simulink model "ASM_Traffic_new"  (R2024a)
settings: Solver=ode1  StartTime=SIM.tstart.v  StopTime=SIM.tend.v  FixedStep=SIM.StepSize.v  RelTol=1e-3
PostLoadFcn:
  | if any(exist('dsrtsu_mdlpostloadfcn', 'file') ~= 0), dsrtsu_mdlpostloadfcn('Execute', bdroot); end
  | try, asm_mdl_postloadfcn(bdroot, 'UpdateModel', 3600); catch, disp(lasterr); end,
InitFcn:
  | , if any(exist('rtifpga_mdlclblib', 'file') ~= 0), rtifpga_mdlclblib('Init', bdroot); end,
  | , if any(exist('dsmpb_private', 'file') ~= 0), dsmpb_private('dsmpb_mdlclblib', 'Init', bdroot); end,
undefined symbols (not defined in the file): _to_, a0b2, ASM_BrakeHydraulics_DemoSystems, ASM_VehicleDynamics_DemoSystems, b98103fe8ad365046cd0, BrakeCircuit, CPT, Crankshaft, DiscIntNeverNeededParam, dsmsi, FinalDriveAssembly, MDL, ModeSignals, Pos_BrakePedal_Maneuver, rad, RefSignals, s_to_rpm, SIM, SoftECU, Suspension, Tire, Transmission
libraries: ASM_Traffic_lib x135, simulink x100, ASM_Utils_lib x77, ASM_VehicleDynamics_lib x70, ASM_Environment_lib x22, dsmpblib x20, dsmsilib x15, MDLD_Utils_lib x10, ASM_BrakeHydraulics_lib x3
(part 37 of 63)

== system ASM_Traffic_new/Environment/GroundTruth/UserInterface/PAR_Plant/Fellow_Vehicles ==
  Interface_In : Inport
  Bus Creator3 : BusCreator  Inputs=10
  Bus Creator4 : BusCreator  Inputs=1
  Bus Selector : BusSelector  OutputSignals=UserSignals_Customized.Fellow1_TurnLights
  Bus Selector1 : BusSelector  OutputSignals=UserSignals_Customized.Fellow2_TurnLights
  Bus Selector10 : BusSelector  OutputSignals=UserSignals_Customized.Fellow11_TurnLights
  Bus Selector11 : BusSelector  OutputSignals=UserSignals_Customized.Fellow12_TurnLights
  Bus Selector12 : BusSelector  OutputSignals=UserSignals_Customized.Fellow13_TurnLights
  Bus Selector13 : BusSelector  OutputSignals=UserSignals_Customized.Fellow14_TurnLights
  Bus Selector14 : BusSelector  OutputSignals=UserSignals_Customized.Fellow15_TurnLights
  Bus Selector15 : BusSelector  OutputSignals=UserSignals_Customized.Fellow16_TurnLights
  Bus Selector16 : BusSelector  OutputSignals=UserSignals_Customized.Fellow17_TurnLights
  Bus Selector17 : BusSelector  OutputSignals=UserSignals_Customized.Fellow18_TurnLights
  Bus Selector18 : BusSelector  OutputSignals=UserSignals_Customized.Fellow19_TurnLights
  Bus Selector19 : BusSelector  OutputSignals=UserSignals_Customized.Fellow20_TurnLights
  Bus Selector2 : BusSelector  OutputSignals=UserSignals_Customized.Fellow3_TurnLights
  Bus Selector20 : BusSelector  OutputSignals=UserSignals_Customized.Fellow21_TurnLights
  Bus Selector21 : BusSelector  OutputSignals=UserSignals_Customized.Fellow22_TurnLights
  Bus Selector22 : BusSelector  OutputSignals=UserSignals_Customized.Fellow23_TurnLights
  Bus Selector23 : BusSelector  OutputSignals=UserSignals_Customized.Fellow24_TurnLights
  Bus Selector24 : BusSelector  OutputSignals=UserSignals_Customized.Fellow25_TurnLights
  Bus Selector25 : BusSelector  OutputSignals=UserSignals_Customized.Fellow26_TurnLights
  Bus Selector26 : BusSelector  OutputSignals=UserSignals_Customized.Fellow27_TurnLights
  Bus Selector27 : BusSelector  OutputSignals=UserSignals_Customized.Fellow28_TurnLights
  Bus Selector28 : BusSelector  OutputSignals=UserSignals_Customized.Fellow29_TurnLights
  Bus Selector29 : BusSelector  OutputSignals=UserSignals_Customized.Fellow30_TurnLights
  Bus Selector3 : BusSelector  OutputSignals=UserSignals_Customized.Fellow4_TurnLights
  Bus Selector3000 : BusSelector  OutputSignals=Traffic.Plant.Traffic_Signals_toEnvironment
  Bus Selector4 : BusSelector  OutputSignals=UserSignals_Customized.Fellow5_TurnLights
  Bus Selector5 : BusSelector  OutputSignals=UserSignals_Customized.Fellow6_TurnLights
  Bus Selector6 : BusSelector  OutputSignals=UserSignals_Customized.Fellow7_TurnLights
  Bus Selector7 : BusSelector  OutputSignals=UserSignals_Customized.Fellow8_TurnLights
  Bus Selector8 : BusSelector  OutputSignals=UserSignals_Customized.Fellow9_TurnLights
  Bus Selector9 : BusSelector  OutputSignals=UserSignals_Customized.Fellow10_TurnLights
  Demux_Fellow_Lightstates : Subsystem
  Lightstates_Fellow1 : Subsystem
  Lightstates_Fellow10 : Subsystem
  Lightstates_Fellow11 : Subsystem
  Lightstates_Fellow12 : Subsystem
  Lightstates_Fellow13 : Subsystem
  Lightstates_Fellow14 : Subsystem
  Lightstates_Fellow15 : Subsystem
  Lightstates_Fellow16 : Subsystem
  Lightstates_Fellow17 : Subsystem
  Lightstates_Fellow18 : Subsystem
  Lightstates_Fellow19 : Subsystem
  Lightstates_Fellow2 : Subsystem
  Lightstates_Fellow20 : Subsystem
  Lightstates_Fellow21 : Subsystem
  Lightstates_Fellow22 : Subsystem
  Lightstates_Fellow23 : Subsystem
  Lightstates_Fellow24 : Subsystem
  Lightstates_Fellow25 : Subsystem
  Lightstates_Fellow26 : Subsystem
  Lightstates_Fellow27 : Subsystem
  Lightstates_Fellow28 : Subsystem
  Lightstates_Fellow29 : Subsystem
  Lightstates_Fellow3 : Subsystem
  Lightstates_Fellow30 : Subsystem
  Lightstates_Fellow4 : Subsystem
  Lightstates_Fellow5 : Subsystem
  Lightstates_Fellow6 : Subsystem
  Lightstates_Fellow7 : Subsystem
  Lightstates_Fellow8 : Subsystem
  Lightstates_Fellow9 : Subsystem
  Mux : Mux  Inputs=MDL.Traffic.MaxNumFellows.v
  Fellow_Vehicles[] : Outport  VectorParamsAs1DForOutWhenUnconnected=off
  wires:
  Bus Selector29/1 -> Lightstates_Fellow30/1(Fellow_Indicator_State[])  "<Fellow30_TurnLights>"
  Bus Selector28/1 -> Lightstates_Fellow29/1(Fellow_Indicator_State[])  "<Fellow29_TurnLights>"
  Bus Selector27/1 -> Lightstates_Fellow28/1(Fellow_Indicator_State[])  "<Fellow28_TurnLights>"
  Bus Selector26/1 -> Lightstates_Fellow27/1(Fellow_Indicator_State[])  "<Fellow27_TurnLights>"
  Bus Selector25/1 -> Lightstates_Fellow26/1(Fellow_Indicator_State[])  "<Fellow26_TurnLights>"
  Bus Selector24/1 -> Lightstates_Fellow25/1(Fellow_Indicator_State[])  "<Fellow25_TurnLights>"
  Bus Selector23/1 -> Lightstates_Fellow24/1(Fellow_Indicator_State[])  "<Fellow24_TurnLights>"
  Bus Selector22/1 -> Lightstates_Fellow23/1(Fellow_Indicator_State[])  "<Fellow23_TurnLights>"
  Bus Selector21/1 -> Lightstates_Fellow22/1(Fellow_Indicator_State[])  "<Fellow22_TurnLights>"
  Bus Selector20/1 -> Lightstates_Fellow21/1(Fellow_Indicator_State[])  "<Fellow21_TurnLights>"
  Bus Selector19/1 -> Lightstates_Fellow20/1(Fellow_Indicator_State[])  "<Fellow20_TurnLights>"
  Bus Selector18/1 -> Lightstates_Fellow19/1(Fellow_Indicator_State[])  "<Fellow19_TurnLights>"
  Bus Selector17/1 -> Lightstates_Fellow18/1(Fellow_Indicator_State[])  "<Fellow18_TurnLights>"
  Bus Selector16/1 -> Lightstates_Fellow17/1(Fellow_Indicator_State[])  "<Fellow17_TurnLights>"
  Bus Selector15/1 -> Lightstates_Fellow16/1(Fellow_Indicator_State[])  "<Fellow16_TurnLights>"
  Bus Selector14/1 -> Lightstates_Fellow15/1(Fellow_Indicator_State[])  "<Fellow15_TurnLights>"
  Bus Selector13/1 -> Lightstates_Fellow14/1(Fellow_Indicator_State[])  "<Fellow14_TurnLights>"
  Bus Selector12/1 -> Lightstates_Fellow13/1(Fellow_Indicator_State[])  "<Fellow13_TurnLights>"
  Bus Selector11/1 -> Lightstates_Fellow12/1(Fellow_Indicator_State[])  "<Fellow12_TurnLights>"
  Bus Selector10/1 -> Lightstates_Fellow11/1(Fellow_Indicator_State[])  "<Fellow11_TurnLights>"
  Bus Selector9/1 -> Lightstates_Fellow10/1(Fellow_Indicator_State[])  "<Fellow10_TurnLights>"
  Bus Selector8/1 -> Lightstates_Fellow9/1(Fellow_Indicator_State[])  "<Fellow9_TurnLights>"
  Bus Selector7/1 -> Lightstates_Fellow8/1(Fellow_Indicator_State[])  "<Fellow8_TurnLights>"
  Bus Selector6/1 -> Lightstates_Fellow7/1(Fellow_Indicator_State[])  "<Fellow7_TurnLights>"
  Bus Selector5/1 -> Lightstates_Fellow6/1(Fellow_Indicator_State[])  "<Fellow6_TurnLights>"
  Bus Selector4/1 -> Lightstates_Fellow5/1(Fellow_Indicator_State[])  "<Fellow5_TurnLights>"
  Bus Selector3/1 -> Lightstates_Fellow4/1(Fellow_Indicator_State[])  "<Fellow4_TurnLights>"
  Bus Selector2/1 -> Lightstates_Fellow3/1(Fellow_Indicator_State[])  "<Fellow3_TurnLights>"
  Bus Selector1/1 -> Lightstates_Fellow2/1(Fellow_Indicator_State[])  "<Fellow2_TurnLights>"
  Bus Selector/1 -> Lightstates_Fellow1/1(Fellow_Indicator_State[])  "<Fellow1_TurnLights>"
  Bus Selector3000/1 -> Bus Selector1/1, Bus Selector2/1, Bus Selector3/1, Bus Selector4/1, Bus Selector5/1, Bus Selector6/1, Bus Selector7/1, Bus Selector8/1, Bus Selector9/1, Bus Selector10/1, Bus Selector11/1, Bus Selector12/1, Bus Selector13/1, Bus Selector14/1, Bus Selector15/1, Bus Selector16/1, Bus Selector17/1, Bus Selector18/1, Bus Selector19/1, Bus Selector20/1, Bus Selector21/1, Bus Selector22/1, Bus Selector23/1, Bus Selector24/1, Bus Selector25/1, Bus Selector26/1, Bus Selector27/1, Bus Selector28/1, Bus Selector29/1, Bus Selector/1  "<Traffic_Signals_toEnvironment>"
  Lightstates_Fellow30/1(Lightstates[]) -> Mux/30
  Lightstates_Fellow29/1(Lightstates[]) -> Mux/29
  Lightstates_Fellow28/1(Lightstates[]) -> Mux/28
  Lightstates_Fellow27/1(Lightstates[]) -> Mux/27
  Lightstates_Fellow26/1(Lightstates[]) -> Mux/26
  Lightstates_Fellow25/1(Lightstates[]) -> Mux/25
  Lightstates_Fellow24/1(Lightstates[]) -> Mux/24
  Lightstates_Fellow23/1(Lightstates[]) -> Mux/23
  Lightstates_Fellow22/1(Lightstates[]) -> Mux/22
  Lightstates_Fellow21/1(Lightstates[]) -> Mux/21
  Lightstates_Fellow20/1(Lightstates[]) -> Mux/20
  Lightstates_Fellow19/1(Lightstates[]) -> Mux/19
  Lightstates_Fellow18/1(Lightstates[]) -> Mux/18
  Lightstates_Fellow17/1(Lightstates[]) -> Mux/17
  Lightstates_Fellow16/1(Lightstates[]) -> Mux/16
  Lightstates_Fellow1/1(Lightstates[]) -> Mux/1
  Lightstates_Fellow2/1(Lightstates[]) -> Mux/2
  Lightstates_Fellow3/1(Lightstates[]) -> Mux/3
  Lightstates_Fellow4/1(Lightstates[]) -> Mux/4
  Lightstates_Fellow5/1(Lightstates[]) -> Mux/5
  Lightstates_Fellow6/1(Lightstates[]) -> Mux/6
  Lightstates_Fellow7/1(Lightstates[]) -> Mux/7
  Lightstates_Fellow8/1(Lightstates[]) -> Mux/8
  Lightstates_Fellow9/1(Lightstates[]) -> Mux/9
  Lightstates_Fellow10/1(Lightstates[]) -> Mux/10
  Lightstates_Fellow11/1(Lightstates[]) -> Mux/11
  Lightstates_Fellow12/1(Lightstates[]) -> Mux/12
  Lightstates_Fellow13/1(Lightstates[]) -> Mux/13
  Lightstates_Fellow14/1(Lightstates[]) -> Mux/14
  Lightstates_Fellow15/1(Lightstates[]) -> Mux/15
  Mux/1 -> Demux_Fellow_Lightstates/1(Fellow_Lightstates[])
  Bus Creator3/1 -> Bus Creator4/1  "Fellow_Vehicles_LightStates"
  Bus Creator4/1 -> Fellow_Vehicles[]/1  "Fellow_Vehicles[]"
  Demux_Fellow_Lightstates/10(Brake_Fellows[]) -> Bus Creator3/10  "Brake_Light[]"
  Demux_Fellow_Lightstates/9(Indicator_State_Fellows[]) -> Bus Creator3/9  "Indicator_State[]"
  Demux_Fellow_Lightstates/6(Rear_Fog_Light_Fellows[]) -> Bus Creator3/6  "Rear_Fog_Light[]"
  Demux_Fellow_Lightstates/5(License_Plate_Illumination_Fellows[]) -> Bus Creator3/5  "License_Plate_Illumination[]"
  Demux_Fellow_Lightstates/1(High_Beam_Fellows[]) -> Bus Creator3/1  "High_Beam[]"
  Demux_Fellow_Lightstates/2(Reversing_Light_Fellows[]) -> Bus Creator3/2  "Reversing_Light[]"
  Demux_Fellow_Lightstates/3(Front_Fog_Light_Fellows[]) -> Bus Creator3/3  "Front_Fog_Light[]"
  Demux_Fellow_Lightstates/4(Head_Light_Fellows[]) -> Bus Creator3/4  "Head_Light[]"
  Demux_Fellow_Lightstates/7(Emergency_Veh_Illu_Fellows[]) -> Bus Creator3/7  "Emergency_Veh_Illu_Fellows[]"
  Demux_Fellow_Lightstates/8(Service_Veh_Illu_Fellows[]) -> Bus Creator3/8  "Service_Veh_Illu_Fellows[]"
  Interface_In/1 -> Bus Selector3000/1

== system ASM_Traffic_new/Environment/GroundTruth/UserInterface/PAR_Plant/HostVehicle_Data_AutomatedDrivingFunction ==
  Interface_In : Inport
  AutomatedDrivingFunction_1 : Subsystem
  AutomatedDrivingFunction_2 : Subsystem
  AutomatedDrivingFunction_3 : Subsystem
  AutomatedDrivingFunction_4 : Subsystem
  Bus Creator : BusCreator  Inputs=4
  HostVehicle_Data_AutomatedDrivingFunction[] : Outport  VectorParamsAs1DForOutWhenUnconnected=off
  wires:
  AutomatedDrivingFunction_3/1(AutomatedDrivingFunction_FCW[]) -> Bus Creator/3  "AutomatedDrivingFunction_FCW[]"
  AutomatedDrivingFunction_2/1(AutomatedDrivingFunction_AEB[]) -> Bus Creator/2  "AutomatedDrivingFunction_AEB[]"
  AutomatedDrivingFunction_4/1(AutomatedDrivingFunction_4[]) -> Bus Creator/4  "AutomatedDrivingFunction_4[]"
  Interface_In/1 -> AutomatedDrivingFunction_1/1(Interface_In), AutomatedDrivingFunction_2/1(Interface_In), AutomatedDrivingFunction_3/1(Interface_In), AutomatedDrivingFunction_4/1(Interface_In)
  Bus Creator/1 -> HostVehicle_Data_AutomatedDrivingFunction[]/1  "HostVehicle_Data_AutomatedDrivingFunction[]"
  AutomatedDrivingFunction_1/1(AutomatedDrivingFunction_ACC[]) -> Bus Creator/1  "AutomatedDrivingFunction_ACC[]"

== system ASM_Traffic_new/Environment/GroundTruth/UserInterface/PAR_Plant/HostVehicle_Data_VehicleBasics ==
  Bus Creator1 : BusCreator  Inputs=2
  Mode_OperatingState[1Stim|2Int] : Constant  Tag=AD:ASM_Sw_SpeedLimit_Source[1Manual|2RoadScenery]  Value=2
  Stim_OperatingState[] : Constant  Tag=AD:ASM_Sw_SpeedLimit_Source[1Manual|2RoadScenery]
      settings: AttributesFormatString=0Unknown\n1Other\n2Sleep\n3Standby\n4Boarding\n5Entertainment\n6Driving\n7Diagnostic
  HostVehicle_Data_VehicleBasics[] : Outport  VectorParamsAs1DForOutWhenUnconnected=off
  wires:
  Mode_OperatingState[1Stim|2Int]/1 -> Bus Creator1/1  "Mode_OperatingState[1Stim|2Int]"
  Stim_OperatingState[]/1 -> Bus Creator1/2  "Stim_OperatingState[]"
  Bus Creator1/1 -> HostVehicle_Data_VehicleBasics[]/1  "HostVehicle_Data_VehicleBasics[]"

== system ASM_Traffic_new/Environment/GroundTruth/UserInterface/PAR_Plant/HostVehicle_Data_VehicleWheels ==
  Axle_Index[] : Constant  Value=[0 0 1 1 2 2]
  Bus Creator1 : BusCreator  Inputs=2
  Wheel_Index[] : Constant  Value=[1 0 1 0 1 0]
  HostVehicle_Data_VehicleWheels[] : Outport  VectorParamsAs1DForOutWhenUnconnected=off
  wires:
  Bus Creator1/1 -> HostVehicle_Data_VehicleWheels[]/1  "HostVehicle_Data_VehicleWheels[]"
  Wheel_Index[]/1 -> Bus Creator1/2  "Wheel_Idx[]"
  Axle_Index[]/1 -> Bus Creator1/1  "Axle_Idx[]"

== system ASM_Traffic_new/Environment/GroundTruth/UserInterface/PAR_Plant/TrafficLight_Counter ==
  Bus Creator : BusCreator  Inputs=4
  TrafficLight_Counter_1 : Subsystem
  TrafficLight_Counter_2 : Subsystem
  TrafficLight_Counter_3 : Subsystem
  TrafficLight_Counter_4 : Subsystem
  TrafficLight_Counter[] : Outport  VectorParamsAs1DForOutWhenUnconnected=off
  wires:
  TrafficLight_Counter_4/1(TrafficLight_Counter_4[]) -> Bus Creator/4  "TrafficLight_Counter_4[]"
  TrafficLight_Counter_3/1(TrafficLight_Counter_3[]) -> Bus Creator/3  "TrafficLight_Counter_3"
  TrafficLight_Counter_2/1(TrafficLight_Counter_2[]) -> Bus Creator/2  "TrafficLight_Counter_2"
  TrafficLight_Counter_1/1(TrafficLight_Counter_1[]) -> Bus Creator/1  "TrafficLight_Counter_1[]"
  Bus Creator/1 -> TrafficLight_Counter[]/1  "TrafficLight_Counter[]"

== system ASM_Traffic_new/Environment/Maneuver/PlantModel/Customize_UserSignals/CustomizedUserSignals ==
  User1[] : Inport
  User2[] : Inport  Port=2
  User3[] : Inport  Port=3
  User4[] : Inport  Port=4
  User5[] : Inport  Port=5
  User6[] : Inport  Port=6
  User7[] : Inport  Port=7
  User8[] : Inport  Port=8
  User9[] : Inport  Port=9
  User10[] : Inport  Port=10
  User11[] : Inport  Port=11
  User12[] : Inport  Port=12
  User13[] : Inport  Port=13
  User14[] : Inport  Port=14
  Gain{1..14} (14 alike) : Gain
  ExternalSegmentEnd_Mode[] : Outport  VectorParamsAs1DForOutWhenUnconnected=off
  ExternalSegmentEnd_Value[] : Outport  Port=2  VectorParamsAs1DForOutWhenUnconnected=off
  ASM_Vehicle_TurnLights[] : Outport  Port=3  VectorParamsAs1DForOutWhenUnconnected=off
  ECU_Commands[] : Outport  Port=4  VectorParamsAs1DForOutWhenUnconnected=off
  Mnv_DataStream_5[] : Outport  Port=5  VectorParamsAs1DForOutWhenUnconnected=off
  Mnv_DataStream_6[] : Outport  Port=6  VectorParamsAs1DForOutWhenUnconnected=off
  Mnv_DataStream_7[] : Outport  Port=7  VectorParamsAs1DForOutWhenUnconnected=off
  Mnv_DataStream_8[] : Outport  Port=8  VectorParamsAs1DForOutWhenUnconnected=off
  Mnv_DoorFL[] : Outport  Port=9  VectorParamsAs1DForOutWhenUnconnected=off
  Mnv_DoorFR[] : Outport  Port=10  VectorParamsAs1DForOutWhenUnconnected=off
  Mnv_DoorRL[] : Outport  Port=11  VectorParamsAs1DForOutWhenUnconnected=off
  Mnv_DoorRR[] : Outport  Port=12  VectorParamsAs1DForOutWhenUnconnected=off
  Mnv_Hood[] : Outport  Port=13  VectorParamsAs1DForOutWhenUnconnected=off
  Mnv_Trunk[] : Outport  Port=14  VectorParamsAs1DForOutWhenUnconnected=off
  wires:
  Gain8/1 -> Mnv_DataStream_8[]/1  "Mnv_DataStream_8[]"
  Gain7/1 -> Mnv_DataStream_7[]/1  "Mnv_DataStream_7[]"
  Gain6/1 -> Mnv_DataStream_6[]/1  "Mnv_DataStream_6[]"
  Gain5/1 -> Mnv_DataStream_5[]/1  "Mnv_DataStream_5[]"
  User8[]/1 -> Gain8/1
  User7[]/1 -> Gain7/1
  User6[]/1 -> Gain6/1
  User5[]/1 -> Gain5/1
  Gain3/1 -> ASM_Vehicle_TurnLights[]/1  "ASM_Vehicle_TurnLights[]"
  User3[]/1 -> Gain3/1
  User2[]/1 -> Gain2/1
  User1[]/1 -> Gain1/1
  Gain4/1 -> ECU_Commands[]/1  "ECU_Commands[]"
  User4[]/1 -> Gain4/1
  Gain2/1 -> ExternalSegmentEnd_Value[]/1  "ExternalSegmentEnd_Value[]"
  Gain1/1 -> ExternalSegmentEnd_Mode[]/1  "ExternalSegmentEnd_Mode[]"
  Gain9/1 -> Mnv_DoorFL[]/1  "Mnv_DoorFL[]"
  User9[]/1 -> Gain9/1
  Gain10/1 -> Mnv_DoorFR[]/1  "Mnv_DoorFR[]"
  User10[]/1 -> Gain10/1
  User11[]/1 -> Gain11/1
  Gain11/1 -> Mnv_DoorRL[]/1  "Mnv_DoorRL[]"
  User12[]/1 -> Gain14/1
  Gain13/1 -> Mnv_Trunk[]/1  "Mnv_Trunk[]"
  User14[]/1 -> Gain13/1
  User13[]/1 -> Gain12/1
  Gain12/1 -> Mnv_Hood[]/1  "Mnv_Hood[]"
  Gain14/1 -> Mnv_DoorRR[]/1  "Mnv_DoorRR[]"

== system ASM_Traffic_new/Environment/Maneuver/PlantModel/ExternalSegmentEnd/Dist_Front_Min ==
  Dist_Front[m] : Inport
  Min : MinMax
  Replace_NoObjectFound1 : Subsystem
      mask Display: disp ('<= 0 --> 1000')
  Out1 : Outport  VectorParamsAs1DForOutWhenUnconnected=off
  wires:
  Dist_Front[m]/1 -> Replace_NoObjectFound1/1(In1)
  Min/1 -> Out1/1
  Replace_NoObjectFound1/1(Out1) -> Min/1

== system ASM_Traffic_new/Environment/Maneuver/PlantModel/ExternalSegmentEnd/Dist_Rear_Min ==
  Dist_Rear[m] : Inport
  Min : MinMax
  Replace_NoObjectFound1 : Subsystem
      mask Display: disp ('<= 0 --> 1000')
  Out1 : Outport  VectorParamsAs1DForOutWhenUnconnected=off
  wires:
  Replace_NoObjectFound1/1(Out1) -> Min/1
  Min/1 -> Out1/1
  Dist_Rear[m]/1 -> Replace_NoObjectFound1/1(In1)

== system ASM_Traffic_new/Environment/Maneuver/PlantModel/ExternalSegmentEnd/SegmentEndTrigger ==
  ExternalSegmentEnd_Mode[] : Inport
  ExternalSegmentEnd_Value[] : Inport  Port=2
  s_Road[m] : Inport  Port=3
  RollRate_Vehicle[deg|s] : Inport  Port=4
  Distance_Front[m] : Inport  Port=5
  Distance_Rear[m] : Inport  Port=6
  Const_0 : Constant  Value=0
  Const_Nr_SegEndModes_Max[] : Constant  Value=4
  Fishhook : Subsystem
  Multiport Switch : MultiPortSwitch  DataPortOrder=Zero-based contiguous  Inputs=5  zeroidx=on  SaturateOnIntegerOverflow=off  InputSameDT=off
  RelOp_DistFrontSmaller : RelationalOperator  Operator=<=  OutDataTypeStr=boolean  InputSameDT=off
  RelOp_DistRearSmaller : RelationalOperator  Operator=<=  OutDataTypeStr=boolean  InputSameDT=off
  RelOp_PosBigger : RelationalOperator  OutDataTypeStr=boolean  InputSameDT=off
  SaturateAndRound : Subsystem
  External_SegmentEnd[0|1] : Outport  VectorParamsAs1DForOutWhenUnconnected=off
  wires:
  Multiport Switch/1 -> External_SegmentEnd[0|1]/1
  RelOp_PosBigger/1 -> Multiport Switch/3
  Const_0/1 -> Multiport Switch/2
  ExternalSegmentEnd_Value[]/1 -> RelOp_PosBigger/2, Fishhook/1(RollRate_Threshold[deg|s]), RelOp_DistRearSmaller/2, RelOp_DistFrontSmaller/2
  s_Road[m]/1 -> RelOp_PosBigger/1
  RollRate_Vehicle[deg|s]/1 -> Fishhook/2(RollRate_Vehicle_CoG[deg|s])
  Fishhook/1(SegmentEnd_Fishhook) -> Multiport Switch/4
  Const_Nr_SegEndModes_Max[]/1 -> SaturateAndRound/2(Max)
  ExternalSegmentEnd_Mode[]/1 -> SaturateAndRound/1(In)
  SaturateAndRound/1(ExternalSegmentEnd_Mode[]) -> Multiport Switch/1
  Distance_Front[m]/1 -> RelOp_DistFrontSmaller/1
  Distance_Rear[m]/1 -> RelOp_DistRearSmaller/1
  RelOp_DistFrontSmaller/1 -> Multiport Switch/5
  RelOp_DistRearSmaller/1 -> Multiport Switch/6

== system ASM_Traffic_new/Environment/Maneuver/UserInterface/DISP_Plant/ASM_Vehicle_TurnLights[] ==
  In1 : Inport
  Out1 : Outport  VectorParamsAs1DForOutWhenUnconnected=off
  wires:
  In1/1 -> Out1/1

== system ASM_Traffic_new/Environment/Maneuver/UserInterface/DISP_Plant/Angle_SteeringWheel_Maneuver[deg] ==
  In1 : Inport
  Out1 : Outport  VectorParamsAs1DForOutWhenUnconnected=off
  wires:
  In1/1 -> Out1/1

== system ASM_Traffic_new/Environment/Maneuver/UserInterface/DISP_Plant/CurrentSegment[] ==
  In1 : Inport
  Out1 : Outport  VectorParamsAs1DForOutWhenUnconnected=off
  wires:
  In1/1 -> Out1/1

== system ASM_Traffic_new/Environment/Maneuver/UserInterface/DISP_Plant/CurrentSequence[] ==
  In1 : Inport
  Out1 : Outport  VectorParamsAs1DForOutWhenUnconnected=off
  wires:
  In1/1 -> Out1/1

== system ASM_Traffic_new/Environment/Maneuver/UserInterface/DISP_Plant/Gear_Maneuver[] ==
  In1 : Inport
  Out1 : Outport  VectorParamsAs1DForOutWhenUnconnected=off
  wires:
  In1/1 -> Out1/1

== system ASM_Traffic_new/Environment/Maneuver/UserInterface/DISP_Plant/LaneIdx_Maneuver[] ==
  In1 : Inport
  Out1 : Outport  VectorParamsAs1DForOutWhenUnconnected=off
  wires:
  In1/1 -> Out1/1

== system ASM_Traffic_new/Environment/Maneuver/UserInterface/DISP_Plant/LatDriver[1LatCtrl|2LatCtrl2] ==
  In1 : Inport
  Out1 : Outport  VectorParamsAs1DForOutWhenUnconnected=off
  wires:
  In1/1 -> Out1/1

== system ASM_Traffic_new/Environment/Maneuver/UserInterface/DISP_Plant/ManeuverState[] ==
  In1 : Inport
  Out1 : Outport  VectorParamsAs1DForOutWhenUnconnected=off
  wires:
  In1/1 -> Out1/1

== system ASM_Traffic_new/Environment/Maneuver/UserInterface/DISP_Plant/ManeuverTime[s] ==
  In1 : Inport
  Out1 : Outport  VectorParamsAs1DForOutWhenUnconnected=off
  wires:
  In1/1 -> Out1/1

== system ASM_Traffic_new/Environment/Maneuver/UserInterface/DISP_Plant/Mode_AccBr[1Stim|2Driver] ==
  In1 : Inport
  Out1 : Outport  VectorParamsAs1DForOutWhenUnconnected=off
  wires:
  In1/1 -> Out1/1

== system ASM_Traffic_new/Environment/Maneuver/UserInterface/DISP_Plant/Mode_AdaptVeloctiyToRoad[1Off|2On] ==
  In1 : Inport
  Out1 : Outport  VectorParamsAs1DForOutWhenUnconnected=off
  wires:
  In1/1 -> Out1/1

== system ASM_Traffic_new/Environment/Maneuver/UserInterface/DISP_Plant/Mode_GearClutch[1Stim|2Driver|3OpenClutch|4RefGear] ==
  In1 : Inport
  Out1 : Outport  VectorParamsAs1DForOutWhenUnconnected=off
  wires:
  In1/1 -> Out1/1

== system ASM_Traffic_new/Environment/Maneuver/UserInterface/DISP_Plant/Mode_LatCtrl[1Pos|2Yaw] ==
  In1 : Inport
  Out1 : Outport  VectorParamsAs1DForOutWhenUnconnected=off
  wires:
  In1/1 -> Out1/1

== system ASM_Traffic_new/Environment/Maneuver/UserInterface/DISP_Plant/Mode_RelativeLane[0CenterLane|1PreferredLane] ==
  In1 : Inport
  Out1 : Outport  VectorParamsAs1DForOutWhenUnconnected=off
  wires:
  In1/1 -> Out1/1

== system ASM_Traffic_new/Environment/Maneuver/UserInterface/DISP_Plant/Mode_SelectorLever[1Stim|2Driver] ==
  In1 : Inport
  Out1 : Outport  VectorParamsAs1DForOutWhenUnconnected=off
  wires:
  In1/1 -> Out1/1

== system ASM_Traffic_new/Environment/Maneuver/UserInterface/DISP_Plant/Mode_TrafficDriver[1Off|2On] ==
  In1 : Inport
  Out1 : Outport  VectorParamsAs1DForOutWhenUnconnected=off
  wires:
  In1/1 -> Out1/1

== system ASM_Traffic_new/Environment/Maneuver/UserInterface/DISP_Plant/Pos_AccPedal_Maneuver[%] ==
  In1 : Inport
  Out1 : Outport  VectorParamsAs1DForOutWhenUnconnected=off
  wires:
  In1/1 -> Out1/1

== system ASM_Traffic_new/Environment/Maneuver/UserInterface/DISP_Plant/Pos_BrakePedal_Maneuver[%] ==
  In1 : Inport
  Out1 : Outport  VectorParamsAs1DForOutWhenUnconnected=off
  wires:
  In1/1 -> Out1/1

== system ASM_Traffic_new/Environment/Maneuver/UserInterface/DISP_Plant/Pos_ClutchPedal_Maneuver[%] ==
  In1 : Inport
  Out1 : Outport  VectorParamsAs1DForOutWhenUnconnected=off
  wires:
  In1/1 -> Out1/1

== system ASM_Traffic_new/Environment/Maneuver/UserInterface/DISP_Plant/Reset_VehicleStates[0|1] ==
  In1 : Inport
  Out1 : Outport  VectorParamsAs1DForOutWhenUnconnected=off
  wires:
  In1/1 -> Out1/1

== system ASM_Traffic_new/Environment/Maneuver/UserInterface/DISP_Plant/RoadControl[] ==
  In1 : Inport
  Out1 : Outport  VectorParamsAs1DForOutWhenUnconnected=off
  wires:
  In1/1 -> Out1/1

== system ASM_Traffic_new/Environment/Maneuver/UserInterface/DISP_Plant/SelectorLever_Maneuver[] ==
  In1 : Inport
  Out1 : Outport  VectorParamsAs1DForOutWhenUnconnected=off
  wires:
  In1/1 -> Out1/1

== system ASM_Traffic_new/Environment/Maneuver/UserInterface/DISP_Plant/d_Maneuver[m] ==
  In1 : Inport
  Out1 : Outport  VectorParamsAs1DForOutWhenUnconnected=off
  wires:
  In1/1 -> Out1/1

== system ASM_Traffic_new/Environment/Maneuver/UserInterface/DISP_Plant/s_local[m] ==
  In1 : Inport
  Out1 : Outport  VectorParamsAs1DForOutWhenUnconnected=off
  wires:
  In1/1 -> Out1/1

== system ASM_Traffic_new/Environment/Maneuver/UserInterface/DISP_Plant/t_local[s] ==
  In1 : Inport
  Out1 : Outport  VectorParamsAs1DForOutWhenUnconnected=off
  wires:
  In1/1 -> Out1/1

== system ASM_Traffic_new/Environment/Maneuver/UserInterface/DISP_Plant/v_Vehicle_Ref_Maneuver[km|h] ==
  In1 : Inport
  Out1 : Outport  VectorParamsAs1DForOutWhenUnconnected=off
  wires:
  In1/1 -> Out1/1

== system ASM_Traffic_new/Environment/Maneuver/UserInterface/DISP_Plant/v_Vehicle_Ref_Maneuver[m|s] ==
  In1 : Inport
  Out1 : Outport  VectorParamsAs1DForOutWhenUnconnected=off
  wires:
  In1/1 -> Out1/1

== system ASM_Traffic_new/Environment/Maneuver/UserInterface/DISP_Plant/v_Vehicle_Ref_Preview_Maneuver[m|s] ==
  In1 : Inport
  Out1 : Outport  VectorParamsAs1DForOutWhenUnconnected=off
  wires:
  In1/1 -> Out1/1

== system ASM_Traffic_new/Environment/Maneuver/UserInterface/DISP_Plant/v_Vehicle_Ref_Preview_State[0Invalid|1CurrentSeg|2NextSeg] ==
  In1 : Inport
  Out1 : Outport  VectorParamsAs1DForOutWhenUnconnected=off
  wires:
  In1/1 -> Out1/1

== system ASM_Traffic_new/Environment/Maneuver/UserInterface/PAR_Plant/Enable_External_Interfaces ==
  Bus Creator2 : BusCreator  Inputs=3
  Sw_AnimationInterface[0Disabled|1Enabled] : Constant  Value=SIM.Sw_AnimationInterface.v
  Sw_ModelDeskPlottingInterface[0Disabled|1Enabled] : Constant  Value=SIM.Sw_ModelDeskPlottingInterface.v
  Sw_ModelPortBlocks[0Disabled|1Enabled] : Constant  Value=SIM.Sw_ModelPortBlocks.v
  Out : Outport
  wires:
  Sw_ModelDeskPlottingInterface[0Disabled|1Enabled]/1 -> Bus Creator2/1  "Sw_ModelDeskPlottingInterface[0Disabled|1Enabled]"
  Sw_ModelPortBlocks[0Disabled|1Enabled]/1 -> Bus Creator2/2  "Sw_ModelPortBlocks[0Disabled|1Enabled]"
  Bus Creator2/1 -> Out/1  "Enable_External_Interfaces"
  Sw_AnimationInterface[0Disabled|1Enabled]/1 -> Bus Creator2/3  "Sw_AnimationInterface[0Disabled|1Enabled]"

== system ASM_Traffic_new/Environment/Maneuver/UserInterface/PAR_Plant/ManeuverControl ==
  Bus Creator : BusCreator  Inputs=4
  Enable_ManeuverStart : Subsystem
      mask Display: disp('Enable ManeuverStart')
  MANEUVER_START : ASM_Utils_lib/ModelDeskInterface/ManeuverControl/MANEUVER_START  Tag=ASM_SUBCOMPONENT  MDLDCtrl_ManeuverStart=0  ASMProperties=struct('Name','MANEUVER_START','Version','3.0','Library','ASM_Utils_lib')  ASMInstanceName=maneuver_start  ASMInstanceID=1
  MANEUVER_STOP : ASM_Utils_lib/ModelDeskInterface/ManeuverControl/MANEUVER_STOP  Tag=ASM_SUBCOMPONENT  MDLDCtrl_ManeuverStop=0  ASMProperties=struct('Name','MANEUVER_STOP','Version','3.0','Library','ASM_Utils_lib')  ASMInstanceName=maneuver_stop  ASMInstanceID=1
  RESET : ASM_Utils_lib/ModelDeskInterface/ManeuverControl/RESET  Tag=ASM_SUBCOMPONENT  MDLDCtrl_Reset=0  ASMProperties=struct('Name','RESET','Version','3.0','Library','ASM_Utils_lib')  ASMInstanceName=reset  ASMInstanceID=1
  Sw_ManualDriving[1ManSched|2Manual] : Constant
  Sw_StartManeuverAtSimStart[0|1] : Constant
  Out1 : Outport  VectorParamsAs1DForOutWhenUnconnected=off
  wires:
  Sw_ManualDriving[1ManSched|2Manual]/1 -> Bus Creator/3  "Sw_ManualDriving[1ManSched|2Manual]"
  Bus Creator/1 -> Out1/1  "Sw_ManeuverControl"
  MANEUVER_STOP/1 -> Bus Creator/2  "ManeuverStop[0|1]"
  RESET/1 -> Bus Creator/4  "Reset[0|1]"
  Sw_StartManeuverAtSimStart[0|1]/1 -> Enable_ManeuverStart/1(Sw_StartManeuverAtSimStart[0|1])
  Enable_ManeuverStart/1(Out) -> Bus Creator/1  "ManeuverStart[0|1]"
  MANEUVER_START/1 -> Enable_ManeuverStart/2(In)

== system ASM_Traffic_new/Environment/Maneuver/UserInterface/PAR_Plant/ManeuverSettings ==
  External_In : Inport
  Bus Creator2 : BusCreator  Inputs=7
  Const_Replace_Pos_BrakePedal[%] : Constant  Value=70
  Pos_BrakePedal_Seg_BrakeUntilStop[%] : Constant  Value=15
  Pos_BrakePedal_Seg_Standstill[%] : Constant  Value=15
  Pos_BrakePedal_State_Brake[%] : Constant  Value=15
  Pos_BrakePedal_State_Wait[%] : Constant  Value=70
  Pos_ClutchPedal_Seg_Standstill[%] : Constant  Value=0
  Rate_Angle_SteeringWheel_State_Wait[deg|s] : Constant  Value=360
  RelOffset_z_Init_Reset_Manual[m] : Constant  Value=0.01
  Replace_BrakePedal_Brake : Subsystem
  Out1 : Outport  VectorParamsAs1DForOutWhenUnconnected=off
  wires:
  Bus Creator2/1 -> Out1/1  "Sw_ManeuverSettings"
  Rate_Angle_SteeringWheel_State_Wait[deg|s]/1 -> Bus Creator2/6  "Rate_Angle_SteeringWheel_State_Wait[deg|s]"
  Pos_BrakePedal_State_Brake[%]/1 -> Replace_BrakePedal_Brake/2(Pos_BrakePedal_Brake[%]_)
  Pos_BrakePedal_State_Wait[%]/1 -> Bus Creator2/3  "Pos_BrakePedal_State_Wait[%]"
  Pos_BrakePedal_Seg_Standstill[%]/1 -> Bus Creator2/4  "Pos_BrakePedal_Seg_Standstill[%]"
  Pos_ClutchPedal_Seg_Standstill[%]/1 -> Bus Creator2/5  "Pos_ClutchPedal_Seg_Standstill[%]"
  Replace_BrakePedal_Brake/1(Pos_BrakePedal_Brake[%]) -> Bus Creator2/1  "Pos_BrakePedal_State_Brake[%]"
  Const_Replace_Pos_BrakePedal[%]/1 -> Replace_BrakePedal_Brake/4(Pos_BrakePedal_Replace[%])
  Replace_BrakePedal_Brake/2(Pos_BrakePedal_BrakeUntilStop[%]) -> Bus Creator2/2  "Pos_BrakePedal_Seg_BrakeUntilStop[%]"
  Pos_BrakePedal_Seg_BrakeUntilStop[%]/1 -> Replace_BrakePedal_Brake/3(Pos_BrakePedal_BrakeUntilStop[%]_)
  RelOffset_z_Init_Reset_Manual[m]/1 -> Bus Creator2/7  "RelOffset_z_Init_Reset_Manual[m]"
  External_In/1 -> Replace_BrakePedal_Brake/1(Sw_MasterBrakeCylinder_Mode[1linear|2physical])

== system ASM_Traffic_new/Environment/Maneuver/UserInterface/PAR_Plant/ManualControl ==
  Angle_SteeringWheel[deg] : Constant  Value=0
  Bus Creator : BusCreator  Inputs=10
  Bus Creator1 : BusCreator  Inputs=3
  Bus Creator2 : BusCreator  Inputs=2
  Bus Creator3 : BusCreator  Inputs=8
  Bus Creator4 : BusCreator  Inputs=3
  Bus Creator5 : BusCreator  Inputs=2
  Bus Creator6 : BusCreator  Inputs=3
  Bus Creator7 : BusCreator  Inputs=1
  Bus Creator8 : BusCreator  Inputs=7
  Const_Steering_Mode_Manual[1Angle|2Trq] : Constant
  EngOpNum[] : Constant  Value=0
  Gear[] : Constant  Value=0
  LaneIdx_Ref[] : Constant  Value=0
  Mode_SelectorLever[1Stim|2Driver] : Constant  Value=2
  Mode_StartButtonState[1Stim|2SoftECU] : Constant  Value=2
  Pos_AccPedal[%] : Constant  Value=0
  Pos_BrakePedal[%] : Constant  Value=0
  Pos_ClutchPedal[%] : Constant  Value=100
  SelectorLever[] : Constant  Value=0
  StarterPermanentOn_Handling : Subsystem
  State_StartButton[-1PowerOff|0Acc|1PowerOn|2StarterOn] : Constant  Value=-1
  Sw_BrakeLight[0Off|1On] : Constant  Value=0
  Sw_DoorFL[0Closed_1Open] : Constant  Value=0
  Sw_DoorFR[0Closed_1Open] : Constant  Value=0
  Sw_DoorRL[0Closed_1Open] : Constant  Value=0
  Sw_DoorRR[0Closed_1Open] : Constant  Value=0
  Sw_Hood[0Closed_1Open] : Constant  Value=0
  Sw_ManualControl_Doors[1Maneuver|2Manual] : Constant
  Sw_ManualControl_Lights[1Maneuver|2Manual] : Constant
  Sw_ParkingBrake[0Off|1On] : Constant  Value=0
  Sw_StartButton[0Off|1On] : Constant  Value=0
  Sw_Starter_PermanentOn[0Off|1On] : Constant
  Sw_Steering_Mode[1Manual|2ManSched] : Constant  Value=2
  Sw_Testbench[0Off|1On] : Constant
  Sw_TipShift[-1Down|0Off|1Up] : Constant  Value=0
  Sw_Trunk[0Closed_1Open] : Constant  Value=0
  Sw_TurnLights[0Off|1Left|2Right|3Both] : Constant  Value=0
  TestBench_Switch : Subsystem
  Trq_Steering[Nm] : Constant  Value=0
  d_Ref[m] : Constant  Value=0
  n_Engine_Testbench_Set[rpm] : Constant  Value=1000
  v_Vehicle_Ref[m|s] : Constant  Value=0
  Out1 : Outport  VectorParamsAs1DForOutWhenUnconnected=off
  wires:
  Sw_Steering_Mode[1Manual|2ManSched]/1 -> Bus Creator5/1  "Sw_Steering_Mode[1Manual|2ManSched]"
  Bus Creator5/1 -> Bus Creator3/6  "Steering"
  Const_Steering_Mode_Manual[1Angle|2Trq]/1 -> Bus Creator5/2  "Const_Steering_Mode_Manual[1Angle|2Trq]"
  SelectorLever[]/1 -> Bus Creator/10  "SelectorLever[]"
  Trq_Steering[Nm]/1 -> Bus Creator/9  "Trq_Steering[Nm]"
  Bus Creator3/1 -> Out1/1  "ManualControl"
  Pos_BrakePedal[%]/1 -> Bus Creator/2  "Pos_BrakePedal[%]"
  Angle_SteeringWheel[deg]/1 -> Bus Creator/5  "Angle_SteeringWheel[deg]"
  v_Vehicle_Ref[m|s]/1 -> Bus Creator/6  "v_Vehicle_Ref[m|s]"
  Gear[]/1 -> Bus Creator/4  "Gear[]"
  Pos_ClutchPedal[%]/1 -> Bus Creator/3  "Pos_ClutchPedal[%]"
  Pos_AccPedal[%]/1 -> Bus Creator/1  "Pos_AccPedal[%]"
  d_Ref[m]/1 -> Bus Creator/7  "d_Ref[m]"
  LaneIdx_Ref[]/1 -> Bus Creator/8  "LaneIdx_Ref[]"
  Bus Creator/1 -> Bus Creator3/1  "ManualDriving"
  Bus Creator2/1 -> Bus Creator3/2  "AutomaticTransmission"
  Sw_TipShift[-1Down|0Off|1Up]/1 -> Bus Creator2/2  "Sw_TipShift[-1Down|0Off|1Up]"
  Mode_SelectorLever[1Stim|2Driver]/1 -> Bus Creator2/1  "Mode_SelectorLever[1Stim|2Driver]"
  Sw_ParkingBrake[0Off|1On]/1 -> Bus Creator7/1  "Sw_ParkingBrake[0Off|1On]"
  Sw_BrakeLight[0Off|1On]/1 -> Bus Creator1/2  "Sw_BrakeLight[0Off|1On]"
  Sw_TurnLights[0Off|1Left|2Right|3Both]/1 -> Bus Creator1/3  "Sw_TurnLights[0Off|1Left|2Right|3Both]"
  Bus Creator1/1 -> Bus Creator3/4  "VehicleLights"
  Sw_ManualControl_Lights[1Maneuver|2Manual]/1 -> Bus Creator1/1  "Sw_ManualControl_Lights[1Maneuver|2Manual]"
  Sw_Starter_PermanentOn[0Off|1On]/1 -> StarterPermanentOn_Handling/3(In3)
  Sw_StartButton[0Off|1On]/1 -> Bus Creator4/1  "Sw_StartButton[0Off|1On]"
  StarterPermanentOn_Handling/1(Out1) -> Bus Creator4/2  "Mode_StartButtonState[1Stim|2SoftECU]"
  Bus Creator4/1 -> Bus Creator3/7  "StartButton"
  StarterPermanentOn_Handling/2(Out2) -> Bus Creator4/3  "State_StartButton[-1PowerOff|0Acc|1PowerOn|2StarterOn]"
  State_StartButton[-1PowerOff|0Acc|1PowerOn|2StarterOn]/1 -> StarterPermanentOn_Handling/2(In2)
  Mode_StartButtonState[1Stim|2SoftECU]/1 -> StarterPermanentOn_Handling/1(In1)
  Sw_Testbench[0Off|1On]/1 -> TestBench_Switch/1(In1)
  TestBench_Switch/1(Out1) -> Bus Creator6/1  "Sw_Testbench[0Off|1On]"
  Bus Creator6/1 -> Bus Creator3/8  "Testbench"
  n_Engine_Testbench_Set[rpm]/1 -> Bus Creator6/3  "n_Engine_Set[rpm]"
  EngOpNum[]/1 -> Bus Creator6/2, TestBench_Switch/2(In2)  "EngOpNum[]"
  Bus Creator7/1 -> Bus Creator3/3  "ParkingBrake"
  Sw_DoorFR[0Closed_1Open]/1 -> Bus Creator8/3  "Sw_DoorFR[0Closed_1Open]"
  Sw_ManualControl_Doors[1Maneuver|2Manual]/1 -> Bus Creator8/1  "Sw_ManualControl_Doors[1Maneuver|2Manual]"
  Bus Creator8/1 -> Bus Creator3/5  "Doors"
  Sw_DoorFL[0Closed_1Open]/1 -> Bus Creator8/2  "Sw_DoorFL[0Closed_1Open]"
  Sw_DoorRL[0Closed_1Open]/1 -> Bus Creator8/4  "Sw_DoorRL[0Closed_1Open]"
  Sw_DoorRR[0Closed_1Open]/1 -> Bus Creator8/5  "Sw_DoorRR[0Closed_1Open]"
  Sw_Trunk[0Closed_1Open]/1 -> Bus Creator8/7  "Sw_Trunk[0Closed_1Open]"
  Sw_Hood[0Closed_1Open]/1 -> Bus Creator8/6  "Sw_Hood[0Closed_1Open]"

== system ASM_Traffic_new/Environment/Maneuver/UserInterface/PAR_Plant/SimulationControl ==
  note: 0 : Do not keep vehicle position at any condition.
      | 1 : Keep vehicle position at special conditions, e.g. if roll/pitch angle exceeds limits (prevents vehicle from falling over).
  Bus Creator : BusCreator  Inputs=2
  Bus Creator1 : BusCreator  Inputs=2
  Max_Angle_Pitch[deg] : Constant  Value=89
  Max_Angle_Roll[deg] : Constant  Value=89
  Sw_Keep_VehiclePosition[0Off|1On] : Constant
  Out1 : Outport  VectorParamsAs1DForOutWhenUnconnected=off
  wires:
  Bus Creator1/1 -> Out1/1  "SimulationControl"
  Sw_Keep_VehiclePosition[0Off|1On]/1 -> Bus Creator1/1  "Sw_Keep_VehiclePosition[0Off|1On]"
  Bus Creator/1 -> Bus Creator1/2  "MaxAngleRollPitch"
  Max_Angle_Roll[deg]/1 -> Bus Creator/1  "Max_Angle_Roll[deg]"
  Max_Angle_Pitch[deg]/1 -> Bus Creator/2  "Max_Angle_Pitch[deg]"

== system ASM_Traffic_new/Environment/Maneuver/UserInterface/PAR_Plant/Vehicle_Inits ==
  Bus Creator2 : BusCreator  Inputs=6
  v_x_Init[km|h] : Constant  Value=0  VectorParams1D=off
  v_y_Init[m|s] : Constant  Value=0  VectorParams1D=off
  v_z_Init[m|s] : Constant  Value=0  VectorParams1D=off
  w_x_Init[rad|s] : Constant  Value=0  VectorParams1D=off
  w_y_Init[rad|s] : Constant  Value=0  VectorParams1D=off
  w_z_Init[rad|s] : Constant  Value=0  VectorParams1D=off
  Out1 : Outport  VectorParamsAs1DForOutWhenUnconnected=off
  wires:
  v_y_Init[m|s]/1 -> Bus Creator2/2  "v_y_Init[km|h]"
  v_z_Init[m|s]/1 -> Bus Creator2/3  "v_z_Init[km|h]"
  w_z_Init[rad|s]/1 -> Bus Creator2/6  "w_z_Init[rad|s]"
  w_y_Init[rad|s]/1 -> Bus Creator2/5  "w_y_Init[rad|s]"
  w_x_Init[rad|s]/1 -> Bus Creator2/4  "w_x_Init[rad|s]"
  v_x_Init[km|h]/1 -> Bus Creator2/1  "v_x_Init[km|h]"
  Bus Creator2/1 -> Out1/1  "Vehicle_Init"

== system ASM_Traffic_new/Environment/Road/PlantModel/Customize_UserSignals/CustomizedUserSignals ==
  User1[] : Inport
  User2[] : Inport  Port=2
  User3[] : Inport  Port=3
  Gain1 : Gain
  Gain2 : Gain
  Gain3 : Gain
  GPS_Method[] : Outport  VectorParamsAs1DForOutWhenUnconnected=off
  Const_Offset_Lat[deg] : Outport  Port=2  VectorParamsAs1DForOutWhenUnconnected=off
  Const_Offset_Long[deg] : Outport  Port=3  VectorParamsAs1DForOutWhenUnconnected=off
  wires:
  Gain1/1 -> GPS_Method[]/1  "GPS_Method[]"
  Gain2/1 -> Const_Offset_Lat[deg]/1  "Const_Offset_Lat[deg]"
  Gain3/1 -> Const_Offset_Long[deg]/1  "Const_Offset_Long[deg]"
  User3[]/1 -> Gain3/1
  User1[]/1 -> Gain1/1
  User2[]/1 -> Gain2/1

== system ASM_Traffic_new/Environment/Road/PlantModel/Customize_UserSignals/User10 ==
  In1 : Inport
  Gain : Gain  SaturateOnIntegerOverflow=on  OutDataTypeStr=Inherit: Same as input  ParamDataTypeStr=Inherit: Same as input
  Out1 : Outport  VectorParamsAs1DForOutWhenUnconnected=off
  wires:
  In1/1 -> Gain/1
  Gain/1 -> Out1/1

== system ASM_Traffic_new/Environment/Road/PlantModel/Customize_UserSignals/User4 ==
  In1 : Inport
  Gain : Gain  SaturateOnIntegerOverflow=on  OutDataTypeStr=Inherit: Same as input  ParamDataTypeStr=Inherit: Same as input
  Out1 : Outport  VectorParamsAs1DForOutWhenUnconnected=off
  wires:
  In1/1 -> Gain/1
  Gain/1 -> Out1/1

== system ASM_Traffic_new/Environment/Road/PlantModel/Customize_UserSignals/User5 ==
  In1 : Inport
  Gain : Gain  SaturateOnIntegerOverflow=on  OutDataTypeStr=Inherit: Same as input  ParamDataTypeStr=Inherit: Same as input
  Out1 : Outport  VectorParamsAs1DForOutWhenUnconnected=off
  wires:
  In1/1 -> Gain/1
  Gain/1 -> Out1/1

== system ASM_Traffic_new/Environment/Road/PlantModel/Customize_UserSignals/User6 ==
  In1 : Inport
  Gain : Gain  SaturateOnIntegerOverflow=on  OutDataTypeStr=Inherit: Same as input  ParamDataTypeStr=Inherit: Same as input
  Out1 : Outport  VectorParamsAs1DForOutWhenUnconnected=off
  wires:
  In1/1 -> Gain/1
  Gain/1 -> Out1/1

== system ASM_Traffic_new/Environment/Road/PlantModel/Customize_UserSignals/User7 ==
  In1 : Inport
  Gain : Gain  SaturateOnIntegerOverflow=on  OutDataTypeStr=Inherit: Same as input  ParamDataTypeStr=Inherit: Same as input
  Out1 : Outport  VectorParamsAs1DForOutWhenUnconnected=off
  wires:
  In1/1 -> Gain/1
  Gain/1 -> Out1/1

== system ASM_Traffic_new/Environment/Road/PlantModel/Customize_UserSignals/User8 ==
  In2 : Inport
  Gain1 : Gain  SaturateOnIntegerOverflow=on  OutDataTypeStr=Inherit: Same as input  ParamDataTypeStr=Inherit: Same as input
  Out2 : Outport  VectorParamsAs1DForOutWhenUnconnected=off
  wires:
  In2/1 -> Gain1/1
  Gain1/1 -> Out2/1

== system ASM_Traffic_new/Environment/Road/PlantModel/Customize_UserSignals/User9 ==
  In2 : Inport
  Gain1 : Gain  SaturateOnIntegerOverflow=on  OutDataTypeStr=Inherit: Same as input  ParamDataTypeStr=Inherit: Same as input
  Out2 : Outport  VectorParamsAs1DForOutWhenUnconnected=off
  wires:
  In2/1 -> Gain1/1
  Gain1/1 -> Out2/1

== system ASM_Traffic_new/Environment/Road/UserInterface/DISP_Plant/Angle_Yaw_Veh_Road[deg] ==
  In1 : Inport
  Out1 : Outport  VectorParamsAs1DForOutWhenUnconnected=off
  wires:
  In1/1 -> Out1/1

== system ASM_Traffic_new/Environment/Road/UserInterface/DISP_Plant/Curv_Veh_Road[1|m] ==
  In1 : Inport
  Out1 : Outport  VectorParamsAs1DForOutWhenUnconnected=off
  wires:
  In1/1 -> Out1/1

== system ASM_Traffic_new/Environment/Road/UserInterface/DISP_Plant/Distance_Marker_Left[m] ==
  In1 : Inport
  Out1 : Outport  VectorParamsAs1DForOutWhenUnconnected=off
  wires:
  In1/1 -> Out1/1

== system ASM_Traffic_new/Environment/Road/UserInterface/DISP_Plant/Distance_Marker_Right[m] ==
  In1 : Inport
  Out1 : Outport  VectorParamsAs1DForOutWhenUnconnected=off
  wires:
  In1/1 -> Out1/1

== system ASM_Traffic_new/Environment/Road/UserInterface/DISP_Plant/Distance_MeasPnt1_Marker_Left[m] ==
  In1 : Inport
  Out1 : Outport  VectorParamsAs1DForOutWhenUnconnected=off
  wires:
  In1/1 -> Out1/1

== system ASM_Traffic_new/Environment/Road/UserInterface/DISP_Plant/Distance_MeasPnt1_Marker_Right[m] ==
  In1 : Inport
  Out1 : Outport  VectorParamsAs1DForOutWhenUnconnected=off
  wires:
  In1/1 -> Out1/1

== system ASM_Traffic_new/Environment/Road/UserInterface/DISP_Plant/Distance_MeasPnt2_Marker_Left[m] ==
  In1 : Inport
  Out1 : Outport  VectorParamsAs1DForOutWhenUnconnected=off
  wires:
  In1/1 -> Out1/1

== system ASM_Traffic_new/Environment/Road/UserInterface/DISP_Plant/Distance_MeasPnt2_Marker_Right[m] ==
  In1 : Inport
  Out1 : Outport  VectorParamsAs1DForOutWhenUnconnected=off
  wires:
  In1/1 -> Out1/1

== system ASM_Traffic_new/Environment/Road/UserInterface/DISP_Plant/Fric_Coeff_CP[:][] ==
  In1 : Inport
  Out1 : Outport  VectorParamsAs1DForOutWhenUnconnected=off
  wires:
  In1/1 -> Out1/1

== system ASM_Traffic_new/Environment/Road/UserInterface/DISP_Plant/GPS_Latitude_Road[deg] ==
  In1 : Inport
  Out1 : Outport  VectorParamsAs1DForOutWhenUnconnected=off
  wires:
  In1/1 -> Out1/1

== system ASM_Traffic_new/Environment/Road/UserInterface/DISP_Plant/GPS_Longitude_Road[deg] ==
  In1 : Inport
  Out1 : Outport  VectorParamsAs1DForOutWhenUnconnected=off
  wires:
  In1/1 -> Out1/1

== system ASM_Traffic_new/Environment/Road/UserInterface/DISP_Plant/LaneWidth[m] ==
  In1 : Inport
  Out1 : Outport  VectorParamsAs1DForOutWhenUnconnected=off
  wires:
  In1/1 -> Out1/1

== system ASM_Traffic_new/Environment/Road/UserInterface/DISP_Plant/MarkerType_Left[] ==
  In1 : Inport
  Out1 : Outport  VectorParamsAs1DForOutWhenUnconnected=off
  wires:
  In1/1 -> Out1/1

== system ASM_Traffic_new/Environment/Road/UserInterface/DISP_Plant/MarkerType_Right[] ==
  In1 : Inport
  Out1 : Outport  VectorParamsAs1DForOutWhenUnconnected=off
  wires:
  In1/1 -> Out1/1

== system ASM_Traffic_new/Environment/Road/UserInterface/DISP_Plant/Pos_x_Ref_Veh_Road[m] ==
  In1 : Inport
  Out1 : Outport  VectorParamsAs1DForOutWhenUnconnected=off
  wires:
  In1/1 -> Out1/1

== system ASM_Traffic_new/Environment/Road/UserInterface/DISP_Plant/Pos_y_Ref_Veh_Road[m] ==
  In1 : Inport
  Out1 : Outport  VectorParamsAs1DForOutWhenUnconnected=off
  wires:
  In1/1 -> Out1/1

== system ASM_Traffic_new/Environment/Road/UserInterface/DISP_Plant/Pos_z_CP[:][m] ==
  In1 : Inport
  Out1 : Outport  VectorParamsAs1DForOutWhenUnconnected=off
  wires:
  In1/1 -> Out1/1

== system ASM_Traffic_new/Environment/Road/UserInterface/DISP_Plant/Slope_Veh_Road[%] ==
  In1 : Inport
  Out1 : Outport  VectorParamsAs1DForOutWhenUnconnected=off
  wires:
  In1/1 -> Out1/1

== system ASM_Traffic_new/Environment/Road/UserInterface/DISP_Plant/Sw_Tire_Parameter_Set_CP[:][1|2|3|4] ==
  In1 : Inport
  Out1 : Outport  VectorParamsAs1DForOutWhenUnconnected=off
  wires:
  In1/1 -> Out1/1

== system ASM_Traffic_new/Environment/Road/UserInterface/DISP_Plant/T_Ambient[degC] ==
  In1 : Inport
  Out1 : Outport  VectorParamsAs1DForOutWhenUnconnected=off
  wires:
  In1/1 -> Out1/1

== system ASM_Traffic_new/Environment/Road/UserInterface/DISP_Plant/Velocity_MeasPnt1_Marker_Left[m|s] ==
  In1 : Inport
  Out1 : Outport  VectorParamsAs1DForOutWhenUnconnected=off
  wires:
  In1/1 -> Out1/1

== system ASM_Traffic_new/Environment/Road/UserInterface/DISP_Plant/Velocity_MeasPnt1_Marker_Right[m|s] ==
  In1 : Inport
  Out1 : Outport  VectorParamsAs1DForOutWhenUnconnected=off
  wires:
  In1/1 -> Out1/1

== system ASM_Traffic_new/Environment/Road/UserInterface/DISP_Plant/Velocity_MeasPnt2_Marker_Left[m|s] ==
  In1 : Inport
  Out1 : Outport  VectorParamsAs1DForOutWhenUnconnected=off
  wires:
  In1/1 -> Out1/1

== system ASM_Traffic_new/Environment/Road/UserInterface/DISP_Plant/Velocity_MeasPnt2_Marker_Right[m|s] ==
  In1 : Inport
  Out1 : Outport  VectorParamsAs1DForOutWhenUnconnected=off
  wires:
  In1/1 -> Out1/1

== system ASM_Traffic_new/Environment/Road/UserInterface/DISP_Plant/p_Ambient[Pa] ==
  In1 : Inport
  Out1 : Outport  VectorParamsAs1DForOutWhenUnconnected=off
  wires:
  In1/1 -> Out1/1

== system ASM_Traffic_new/Environment/Road/UserInterface/DISP_Plant/s_Veh_Road[m] ==
  In1 : Inport
  Out1 : Outport  VectorParamsAs1DForOutWhenUnconnected=off
  wires:
  In1/1 -> Out1/1

== system ASM_Traffic_new/Environment/Road/UserInterface/PAR_Plant/BasicRoad ==
  Pos_CP_CoorSys_E[:][x;y][m] : Inport
  Bus Creator : BusCreator  Inputs=4
  Fric_Coeff_BasicRoad[] : Constant
  Product : Product
  Product1 : Product
  Slope_BasicRoad[%] : Constant  Value=0
  Slope_Lateral_BasicRoad[deg] : Constant  Value=0
  Subsystem : Subsystem
  Sw_Tire_Parameter_Set[1|2|3|4] : Constant
  Out1 : Outport  VectorParamsAs1DForOutWhenUnconnected=off
  wires:
  Pos_CP_CoorSys_E[:][x;y][m]/1 -> Subsystem/1(Pos_CP_CoorSys_E[:][x;y][m])
  Subsystem/1(Out1) -> Product1/2, Product/2
  Product1/1 -> Bus Creator/4  "Sw_Tire_Parameter_Set_CP_BasicRoad[:][1|2|3|4]"
  Sw_Tire_Parameter_Set[1|2|3|4]/1 -> Product1/1
  Product/1 -> Bus Creator/3  "Fric_Coeff_CP_BasicRoad[:][]"
  Fric_Coeff_BasicRoad[]/1 -> Product/1
  Slope_Lateral_BasicRoad[deg]/1 -> Bus Creator/2  "Slope_Lateral_BasicRoad[deg]"
  Slope_BasicRoad[%]/1 -> Bus Creator/1  "Slope_BasicRoad[%]"
  Bus Creator/1 -> Out1/1  "Sw_BasicRoad"

== system ASM_Traffic_new/Environment/Road/UserInterface/PAR_Plant/Objects_DataStreams ==
  In1 : Inport
  Bus Creator : BusCreator  Inputs=8
  DataStream_1 : Subsystem
  DataStream_2 : Subsystem
  DataStream_3 : Subsystem
  DataStream_4 : Subsystem
  DataStream_5 : Subsystem
  DataStream_6 : Subsystem
  DataStream_7 : Subsystem
  DataStream_8 : Subsystem
  Out1 : Outport  VectorParamsAs1DForOutWhenUnconnected=off
  wires:
  DataStream_8/1(DataStream_8[]) -> Bus Creator/8  "DataStream_8[]"
  DataStream_7/1(DataStream_7[]) -> Bus Creator/7  "DataStream_7[]"
  DataStream_6/1(DataStream_6[]) -> Bus Creator/6  "DataStream_6[]"
  DataStream_5/1(DataStream_5[]) -> Bus Creator/5  "DataStream_5[]"
  DataStream_4/1(DataStream_4[]) -> Bus Creator/4  "DataStream_4[]"
  DataStream_3/1(DataStream_3[]) -> Bus Creator/3  "DataStream_3[]"
  DataStream_2/1(DataStream_2[]) -> Bus Creator/2  "DataStream_2[]"
  DataStream_1/1(DataStream_1[]) -> Bus Creator/1  "DataStream_1[]"
  In1/1 -> DataStream_1/1(Maneuver_Signals[]), DataStream_2/1(Maneuver_Signals[]), DataStream_3/1(Maneuver_Signals[]), DataStream_4/1(Maneuver_Signals[]), DataStream_8/1(Maneuver_Signals[]), DataStream_7/1(Maneuver_Signals[]), DataStream_6/1(Maneuver_Signals[]), DataStream_5/1(Maneuver_Signals[])
  Bus Creator/1 -> Out1/1  "Objects_DataStreams[]"
